simulink model "demoNavalVesselMano"  (R2022a)
settings: Solver=ode45  StartTime=0.0  StopTime=200  RelTol=1e-5  EnableMultiTasking=on
undefined symbols (not defined in the file): magnitude
libraries: mssSimulink x7, simulink x1
settings Model: Creator=thor  LastModifiedBy=thor
settings SolverCC: AlgebraicLoopSolver=TrustRegion
settings DataIOCC: LimitDataPoints=on  SaveFormat=Array  SignalLoggingSaveFormat=ModelDataLogs  ReturnWorkspaceOutputs=off
settings OptimizationCC: InitFltsAndDblsToZero=on  LifeSpan=inf
settings DebuggingCC: SaveWithParameterizedLinksMsg=none  UnderspecifiedInitializationDetection=Classic  MergeDetectMultiDrivingBlocksExec=none  SignalResolutionControl=TryResolveAllWithWarning  MultiTaskDSMMsg=warning  MultiTaskCondExecSysMsg=none  FcnCallInpInsideContextMsg=warning  UnconnectedInputMsg=warning  UnconnectedOutputMsg=warning  UnconnectedLineMsg=warning  SFUnexpectedBacktrackingDiag=warning  SFNoUnconditionalDefaultTransitionDiag=warning  SFExecutionAtInitializationDiag=none  SFMachineParentedDataDiag=warning  ArithmeticOperatorsInVariantConditions=warning
settings HardwareCC: ProdBitPerPointer=32  ProdBitPerSizeT=32  ProdBitPerPtrDiffT=32  ProdLargestAtomicFloat=None  ProdIntDivRoundTo=Undefined  ProdEndianess=Unspecified  ProdWordSize=32  ProdHWDeviceType=32-bit Generic
settings ModelReferenceCC: PropagateSignalLabelsOutOfModel=off
settings SFSimCC: SimUseLocalCustomCode=off  CustomCodeUndefinedFunction=UseInterfaceOnly
settings RTWCC: RTWUseLocalCustomCode=off  DLArmComputeVersion=19.05
settings CodeAppCC: StateflowObjectComments=on
settings GRTTargetCC: TargetFcnLib=ansi_tfl_tmw.mat  TargetLangStandard=C89/C90 (ANSI)  CombineOutputUpdateFcns=off  GRTInterface=on
settings ConfigComp: CovMetricSettings=dw  CovSaveCumulativeToWorkspaceVar=on  CovSaveSingleToWorkspaceVar=on  CovExternalEMLEnable=off

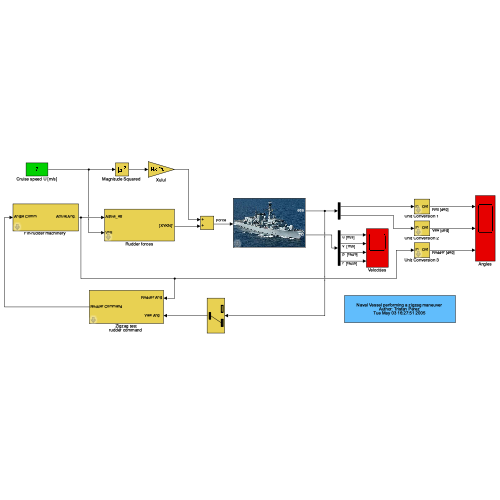
[thumbnail: Simulink's stored preview of the top-level diagram]
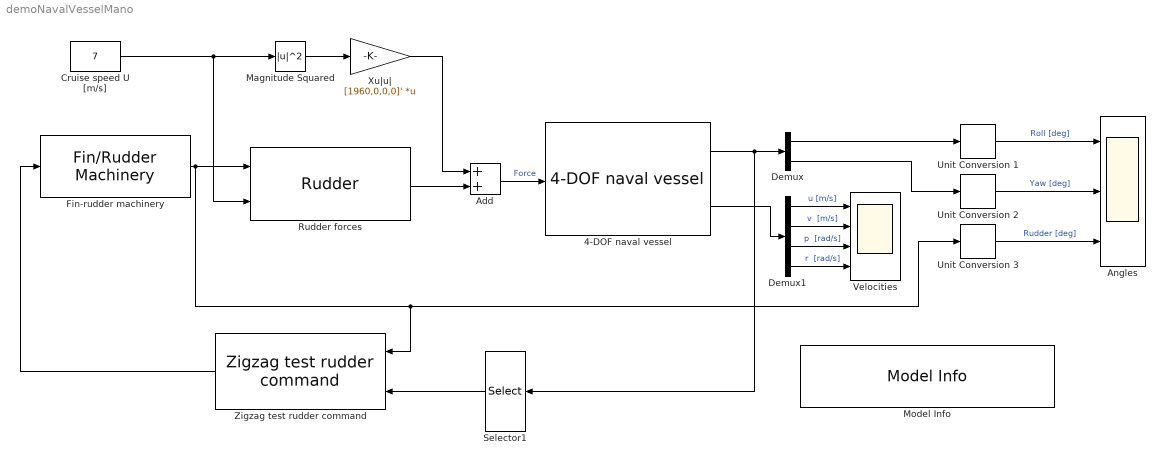
== system demoNavalVesselMano ==
  4-DOF naval vessel : mssSimulink/Marine craft models/4-DOF naval vessel  x0=[7,0,0,0,0,0]'
  Add : Sum
  Angles : Scope  NumInputPorts=3
  Cruise speed U [m/s] : Constant  Value=7
  Demux : Demux  Outputs=2
  Demux1 : Demux
  "Fin-rudder machinery " : mssSimulink/Modelling/Control Surfaces/Fin//Rudder Machinery  Dmax=(pi*45/180)  Dvmax=(pi*20/180)  tc=0.2
  "Magnitude Squared " : Math  Operator=magnitude^2
  Model Info : simulink/Model-Wide Utilities/Model Info  Frame=on  DisplayStringWithTags=|  HorizontalTextAlignment=Center  LeftAlignmentValue=0.5
      | Naval Vessel performing a zigzag maneuver
      | Author: Tristan Perez
      | %<Created>
  Rudder forces : mssSimulink/Modelling/Control Surfaces/Rudder  LCG=19.82  VCG=3.36  sp=1.5  ar=3  A=2*1.5  dCL=1.25/(pi*23/180)  CD0=0.0065  stall=(pi*23/180)  rho=1025
  Selector1 : Selector  InputPortWidth=2  IndexOptions=Index vector (dialog)  Indices=[2]  OutputSizes=1
  Unit Conversion 1 : mssSimulink/Utilities/Math Operations/Unit Conversion  in=rad2deg
  Unit Conversion 2 : mssSimulink/Utilities/Math Operations/Unit Conversion  in=rad2deg
  Unit Conversion 3 : mssSimulink/Utilities/Math Operations/Unit Conversion  in=rad2deg
  Velocities : Scope  NumInputPorts=4
  Xu|u| : Gain  Gain=[1960,0,0,0]'  Multiplication=Matrix(K*u)
  "Zigzag test rudder command " : mssSimulink/Guidance/Zigzag test rudder command   RL=pi*45/180
  wires:
  "Fin-rudder machinery "/1 -> Rudder forces/1, "Zigzag test rudder command "/1, Unit Conversion 3/1
  "Zigzag test rudder command "/1 -> "Fin-rudder machinery "/1
  Selector1/1 -> "Zigzag test rudder command "/2
  4-DOF naval vessel/1 -> Selector1/1, Demux/1
  Add/1 -> 4-DOF naval vessel/1  "Force"
  Rudder forces/1 -> Add/2
  "Magnitude Squared "/1 -> Xu|u|/1
  Xu|u|/1 -> Add/1
  Cruise speed U [m/s]/1 -> "Magnitude Squared "/1, Rudder forces/2
  Demux1/1 -> Velocities/1  "u [m/s]"
  4-DOF naval vessel/2 -> Demux1/1
  Demux1/2 -> Velocities/2  "v  [m/s]"
  Demux1/3 -> Velocities/3  "p  [rad/s]"
  Demux1/4 -> Velocities/4  "r  [rad/s]"
  Unit Conversion 1/1 -> Angles/1  "Roll [deg]"
  Demux/1 -> Unit Conversion 1/1
  Unit Conversion 2/1 -> Angles/2  "Yaw [deg]"
  Unit Conversion 3/1 -> Angles/3  "Rudder [deg]"
  Demux/2 -> Unit Conversion 2/1
